simulink model "FSM_dc_drive"  (R2024a)
settings: Solver=FixedStepDiscrete  StartTime=0.0  StopTime=inf  FixedStep=1e-3  RelTol=1e-3  EnableMultiTasking=on
libraries: arduinolib x2, simulink x2
settings Model: ExtModeTrigDuration=2  Creator=VICTUS  LastModifiedBy=MANSY
settings SolverCC: AutoInsertRateTranBlk=on
settings OptimizationCC: EnhancedBackFolding=on  PassReuseOutputArgsAs=Individual arguments  ZeroExternalMemoryAtStartup=off  ZeroInternalMemoryAtStartup=off  MaxStackSize=64  OptimizeBlockOrder=speed  DifferentSizesBufferReuse=on  OptimizationCustomize=off  EfficientTunableParamExpr=on
settings DebuggingCC: ParameterTunabilityLossMsg=error
settings HardwareCC: ProdBitPerPointer=32  ProdBitPerSizeT=32  ProdBitPerPtrDiffT=32  ProdLargestAtomicInteger=Long  ProdLargestAtomicFloat=Double  ProdWordSize=32  ProdHWDeviceType=ARM Compatible->ARM Cortex
settings SFSimCC: MATLABDynamicMemAlloc=off
settings RTWCC: Description=Embedded Coder  SystemTargetFile=ert.tlc  HardwareBoard=ESP32-WROOM(Arduino Compatible)  TLCOptions="-aInlineSetEventsForThisBaseRateFcn=TLC_FALSE -aSuppressMultiTaskScheduler=TLC_FALSE  -aRateBasedStepFcn=0"  TemplateMakefile=ert_default_tmf  Toolchain=ESP32  BuildConfiguration=Faster Runs
settings CodeAppCC: ForceParamTrailComments=on  IgnoreCustomStorageClasses=off  OperatorAnnotations=on  SimulinkDataObjDesc=on  SFDataObjDesc=on  InsertBlockDesc=on
settings ERTTargetCC: SupportContinuousTime=on  SupportVariableSizeSignals=on  ExtModeTransport=3  ExtModeStaticAlloc=on  ExtModeAutomaticAllocSize=off  ExtModeStaticAllocSize=65536  ExtModeMexFile=ext_xcp  ExtModeIntrfLevel=Level2 - Open

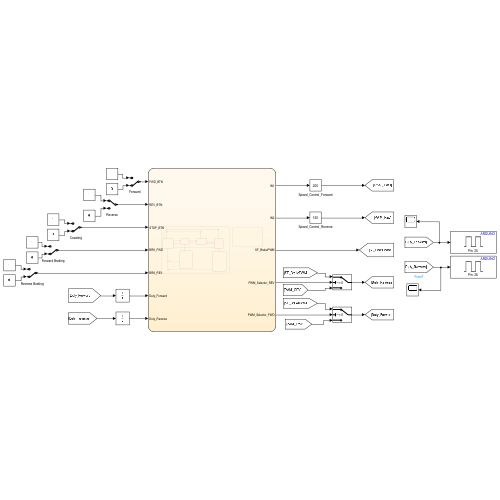
[thumbnail: Simulink's stored preview of the top-level diagram]
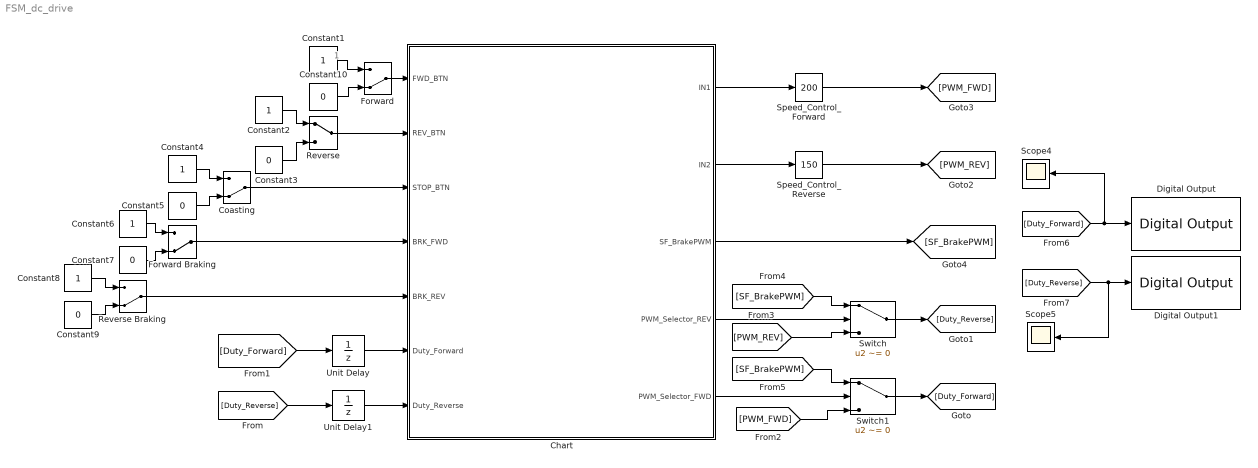
== system FSM_dc_drive ==
  note: 1
  Chart : Stateflow chart  TreatAsAtomicUnit=on
  Coasting : ManualSwitch  CurrentSetting=0
  Constant{1..2,4,6,8} (5 alike) : Constant
  Constant{3,5,7,9..10} (5 alike) : Constant  Value=0
  Digital Output : arduinolib/Digital Output  pinNumber=25  Direction=output  blockPlatform=arduino
  Digital Output1 : arduinolib/Digital Output  pinNumber=26  Direction=output  blockPlatform=arduino
  Forward : ManualSwitch  CurrentSetting=0
  Forward Braking : ManualSwitch  CurrentSetting=0
  Reverse : ManualSwitch
  Reverse Braking : ManualSwitch  CurrentSetting=0
  Scope4 : Scope
  Scope5 : Scope
  Speed_Control_Forward : simulink/Math Operations/Slider Gain  gain=200  low=0  high=255
  Speed_Control_Reverse : simulink/Math Operations/Slider Gain  gain=150  low=0  high=255
  Switch : Switch  Criteria=u2 ~= 0  SaturateOnIntegerOverflow=off  InputSameDT=off
  Switch1 : Switch  Criteria=u2 ~= 0  SaturateOnIntegerOverflow=off  InputSameDT=off
  Unit Delay : UnitDelay  SampleTime=-1  HasFrameUpgradeWarning=on
  Unit Delay1 : UnitDelay  SampleTime=-1  HasFrameUpgradeWarning=on
  wires:
  Forward/1 -> Chart/1(FWD_BTN)
  Coasting/1 -> Chart/3(STOP_BTN)
  Constant2/1 -> Reverse/1
  Constant3/1 -> Reverse/2
  Reverse/1 -> Chart/2(REV_BTN)
  Chart/2(IN2) -> Speed_Control_Reverse/1
  Forward Braking/1 -> Chart/4(BRK_FWD)
  Reverse Braking/1 -> Chart/5(BRK_REV)
  Switch/1 -> [Duty_Reverse]
  Chart/4(PWM_Selector_REV) -> Switch/2
  Chart/1(IN1) -> Speed_Control_Forward/1
  [Duty_Forward] -> Unit Delay/1
  Unit Delay/1 -> Chart/6(Duty_Forward)
  Chart/5(PWM_Selector_FWD) -> Switch1/2
  Switch1/1 -> [Duty_Forward]
  Speed_Control_Forward/1 -> [PWM_FWD]
  Unit Delay1/1 -> Chart/7(Duty_Reverse)
  [Duty_Reverse] -> Unit Delay1/1
  [PWM_FWD] -> Switch1/3
  Speed_Control_Reverse/1 -> [PWM_REV]
  [PWM_REV] -> Switch/3
  Chart/3(SF_BrakePWM) -> [SF_BrakePWM]
  [SF_BrakePWM] -> Switch/1
  [SF_BrakePWM] -> Switch1/1
  [Duty_Forward] -> Scope4/1, Digital Output/1
  [Duty_Reverse] -> Digital Output1/1, Scope5/1
  Constant10/1 -> Forward/2
  Constant1/1 -> Forward/1
  Constant4/1 -> Coasting/1
  Constant5/1 -> Coasting/2
  Constant7/1 -> Forward Braking/2
  Constant6/1 -> Forward Braking/1
  Constant8/1 -> Reverse Braking/1
  Constant9/1 -> Reverse Braking/2

== stateflow chart FSM_dc_drive/Chart ==
  settings: updateMethod=DISCRETE  sampleTime=10e-3
  state Motor_States [parallel]
    settings: executionOrder=2
    state DeadTime
      entry:
      IN1 = 0;
      IN2 = 0;
    state Reverse_Run_Q3
      entry:
      PrevDir = -1;
      IN1 = 0;
      IN2 = 1;
    state Coast_Idle
      entry:
      IN1 = 0;
      IN2 = 0;
    state Forward_Run_Q1
      entry:
      PrevDir = 1;
      IN1 = 1;
      IN2 = 0;
    state Forward_BRK_Q2
      entry:
      brake_spd = Duty_Forward;
      IN1 = 0;
      IN2 = 1;
      PWM_Selector_REV = 1;
      during:
      if brake_spd > 5
      brake_spd = brake_spd - 5;
      else
      brake_spd = 0;
      end
      SF_BrakePWM = brake_spd;
      exit:
      SF_BrakePWM = 0;
      IN2 = 0;
      PWM_Selector_REV = 0;
    state Reverse_BRK_Q4
      entry:
      brake_spd = Duty_Reverse ;
      IN1 = 1;
      IN2 = 0;
      PWM_Selector_FWD = 1;
      during:
      if brake_spd > 5
      brake_spd = brake_spd - 5;
      else
      brake_spd = 0;
      end
      SF_BrakePWM = brake_spd;
      exit:
      SF_BrakePWM = 0;
      IN2 = 0;
      PWM_Selector_FWD = 0;
    (junction 71) -> (junction 79)
    (junction 79) -> (junction 19)
    Reverse_Run_Q3 -> (junction 71) [order 2] : [TargetDir == 0]
    (junction 18) -> (junction 19) : [TargetDir == 0]
    (default) -> Coast_Idle
    (junction 19) -> Coast_Idle
    DeadTime -> (junction 18) [order 1]
    Forward_Run_Q1 -> DeadTime [order 3] : [TargetDir ==  -1&& PrevDir == 1]
    Coast_Idle -> Forward_Run_Q1 [order 1] : [TargetDir == 1]
    DeadTime -> Reverse_Run_Q3 [order 2] : after(30,msec)[TargetDir == -1 && PrevDir== 1]
    DeadTime -> Forward_Run_Q1 [order 3] : [TargetDir == 1]
    Forward_Run_Q1 -> Coast_Idle [order 2] : [TargetDir == 0]
    Reverse_Run_Q3 -> DeadTime [order 3] : [TargetDir == 1]
    Forward_Run_Q1 -> Forward_BRK_Q2 [order 1] : [TargetDir == 2]
    Coast_Idle -> Reverse_Run_Q3 [order 2] : [TargetDir == -1]
    Reverse_Run_Q3 -> Reverse_BRK_Q4 [order 1] : [TargetDir == 3]
    (junction 107) -> Coast_Idle
    Forward_BRK_Q2 -> (junction 107) : [ brake_spd == 0]
    (junction 113) -> (junction 107)
    Reverse_BRK_Q4 -> (junction 113) : [ brake_spd == 0]
  state Input_Logic [parallel]
    entry:
    TargetDir = 0;
    during:
    if(BRK_FWD)
    TargetDir = 2;
    end;
    if(BRK_REV)
    TargetDir = 3;
    end;
    if(STOP_BTN && ~BRK_FWD && ~BRK_REV)
    TargetDir = 0;
    end;
    if (FWD_BTN && ~REV_BTN && ~STOP_BTN && ~BRK_FWD&& ~BRK_REV)
    TargetDir = 1;
    end;
    if (REV_BTN && ~FWD_BTN && ~STOP_BTN&&~BRK_FWD&& ~BRK_REV)
    TargetDir = -1;
    end;
    settings: executionOrder=1
  data: FWD_BTN input; REV_BTN input; STOP_BTN input; IN1 output; IN2 output; BRK_FWD input; BRK_REV input; TargetDir local double; PrevDir local double; brake_spd local; SF_BrakePWM output; PWM_Selector_REV output; Duty_Forward input; PWM_Selector_FWD output; Duty_Reverse input
